simulink model "InvPendIdentPiMod2"  (R2025b)
settings: Solver=ode1  StartTime=0.0  StopTime=40  FixedStep=0.001  RelTol=1e-3
model workspace (MAT data in the model file):
  PID1D = 2
  PID1DD = 2
  PID1DI = 0.1
  PID1DP = 20
  PID1I = 0.1
  PID1P = 7
  PIDD = 2
  PIDDD = 2
  PIDDI = 0.1
  PIDDP = 7
  PIDI = 0.1
  PIDP = 20
undefined symbols (not defined in the file): magnitude, MQTTsample
libraries: simulink x6, slpidlib x4, raspberrypiCommlib x2, raspberrypiBasiclib x1, raspberrypiIOTlib x1
settings Model: SimulationMode=external  ExtModeTrigMode=oneshot  ExtModeTrigDuration=100000  Creator=Administrator  LastModifiedBy=brfon_9d4n8nc
settings SolverCC: AlgebraicLoopSolver=TrustRegion  PositivePriorityOrder=on  AutoInsertRateTranBlk=on
settings DataIOCC: SaveFormat=Array  SignalLoggingSaveFormat=ModelDataLogs  ReturnWorkspaceOutputs=off  SignalLoggingName=sigsOut
settings OptimizationCC: BlockReduction=off  BooleanDataType=off  EnhancedBackFolding=on  PassReuseOutputArgsAs=Individual arguments  ExpressionDepthLimit=2147483647.0  ZeroExternalMemoryAtStartup=off  ZeroInternalMemoryAtStartup=off  InitFltsAndDblsToZero=on  MaxStackSize=200000  OptimizeBlockOrder=speed  DifferentSizesBufferReuse=on  OptimizationCustomize=off  EfficientTunableParamExpr=on
settings DebuggingCC: SaveWithParameterizedLinksMsg=none  UnderspecifiedInitializationDetection=Classic  MergeDetectMultiDrivingBlocksExec=none  SignalResolutionControl=TryResolveAllWithWarning  MultiTaskDSMMsg=warning  ParameterTunabilityLossMsg=error  FcnCallInpInsideContextMsg=warning  UnconnectedInputMsg=warning  UnconnectedOutputMsg=warning  UnconnectedLineMsg=warning  AllowSymbolicDim=off  StateNameClashWarn=warning  SFUnexpectedBacktrackingDiag=warning  SFNoUnconditionalDefaultTransitionDiag=warning  SFExecutionAtInitializationDiag=none  ArithmeticOperatorsInVariantConditions=warning
settings HardwareCC: ProdBitPerLong=64.0  ProdLargestAtomicInteger=LongLong  ProdLargestAtomicFloat=Double  ProdLongLongMode=on  ProdHWDeviceType=ARM Compatible->ARM Cortex-A (64-bit)  TargetBitPerLong=64.0  TargetBitPerPointer=64.0  TargetIntDivRoundTo=Zero  TargetEndianess=LittleEndian  TargetWordSize=64.0  TargetHWDeviceType=Intel->x86-64
settings ModelReferenceCC: EnableRefExpFcnMdlSchedulingChecks=on  PropagateSignalLabelsOutOfModel=off
settings SFSimCC: SimUseLocalCustomCode=off  CustomCodeUndefinedFunction=UseInterfaceOnly
settings RTWCC: SystemTargetFile=ert.tlc  HardwareBoard=Raspberry Pi (64bit)  TLCOptions="-aInlineSetEventsForThisBaseRateFcn=TLC_FALSE -aSuppressMultiTaskScheduler=TLC_FALSE  -aRateBasedStepFcn=0"  TemplateMakefile=ert_default_tmf  RTWUseLocalCustomCode=off  Toolchain=GNU GCC Embedded Linux  BuildConfiguration=Faster Runs  GPUComputeCapability=3.5  Description=Embedded Coder
settings CodeAppCC: ForceParamTrailComments=on  IgnoreCustomStorageClasses=off  MaxIdLength=95.0  OperatorAnnotations=on  SimulinkDataObjDesc=on  SFDataObjDesc=on  InsertBlockDesc=on
settings ERTTargetCC: ExtModeTransport=2.0  ExtModeStaticAlloc=on  ExtModeMexFile=ext_xcp  ExtModeIntrfLevel=Level2 - Open  InlinedParameterPlacement=Hierarchical  CodeReplacementLibrary=ARM Cortex-A CMSIS  SupportContinuousTime=on  SupportVariableSizeSignals=on
settings ConfigComp: CovMetricSettings=dw  CovSaveCumulativeToWorkspaceVar=on  CovSaveSingleToWorkspaceVar=on  CovExternalEMLEnable=off

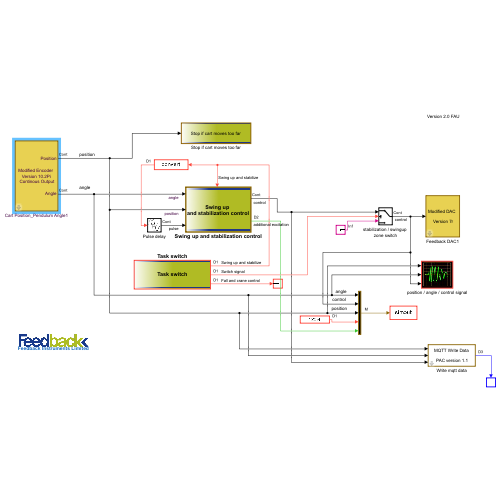
[thumbnail: Simulink's stored preview of the top-level diagram]
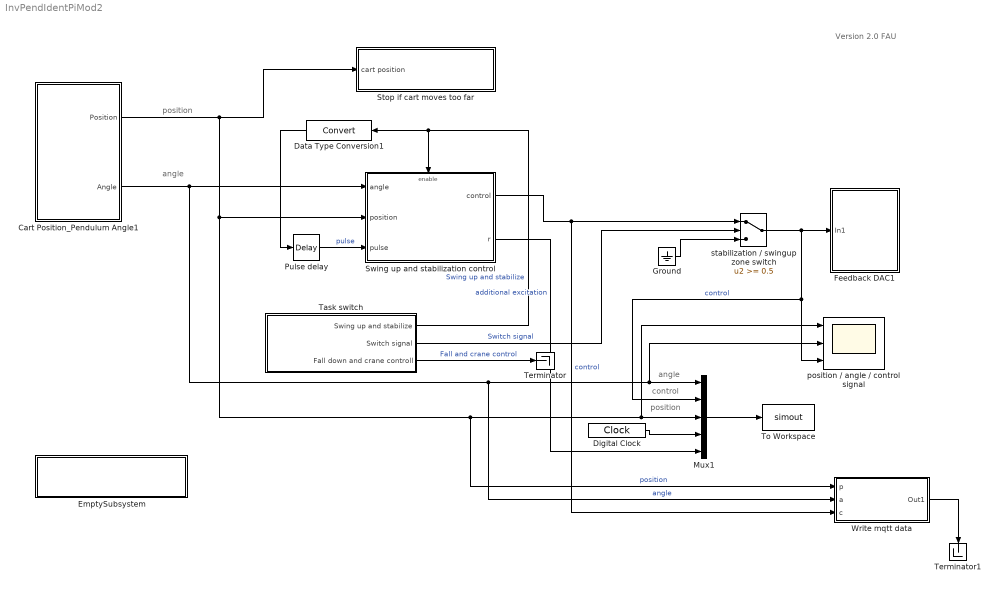
== system InvPendIdentPiMod2 ==
  note: position
  note: angle
  note: Version 2.0 FAU
  note: angle
  note: position
  note: control
  Cart Position_Pendulum Angle1 : Subsystem  mask(Feedback Encoder Block){st=0.001, of1=0, of2=-1024}
      mask prompts: st "Sample Time"; of1 "Channel 1 Offset"; of2 "Channel 2 Offset"
      mask help: Special block to use with the Feedback experiments to read encoder channels using the digital I/O lines
      mask Display:
      | %image(imread('bckg.bmp'))
      | disp('Modified Encoder \nVersion 10.2Pi\n Continous Output')
      | port_label('output', 1, 'Position')
      | port_label('output', 2, 'Angle')
  Data Type Conversion1 : DataTypeConversion  SaturateOnIntegerOverflow=off  RndMeth=Floor
  Digital Clock : DigitalClock  SampleTime=0.001
  EmptySubsystem : Subsystem
      mask Display:
      | image(imread('FB-inst-blue2.jpg'))
      | disp('\n\nFeedback Instruments Limited')
  Feedback DAC1 : Subsystem  mask(DAC Unit for Feedback Experiments){st=0.001, ch=1}
      mask prompts: st "Sample Time"; ch "Output Channel"
      mask help:
      | Digital to Analog Output  for Feedback Experiments
      | using Advantech PCI1711  I/O board
      mask Display:
      | %image(imread('bckg.bmp'))
      | disp('Modified DAC \n\n Version 7r')
  Ground : Ground
  Mux1 : Mux  Inputs=5
  Pulse delay : TransportDelay  DelayTime=0.3  FixedBuffer=on
  Stop if cart moves too far : Subsystem
      mask Display:
      | image(imread('bckg.bmp'))
      | disp('Stop if cart moves too far')
  Swing up and stabilization control : Subsystem  TreatAsAtomicUnit=on
      mask Display:
      | image(imread('bckg.bmp'))
      | disp('Swing up \nand stabilization control')
  Task switch : Subsystem
      mask Display:
      | image(imread('bckg.bmp'))
      | disp('Task switch')
  Terminator : Terminator
  Terminator1 : Terminator
  To Workspace : ToWorkspace  VariableName=simout  SampleTime=0.001
  Write mqtt data : Subsystem
      mask Display: disp('MQTT Write Data\n\n PAC version 1.1')
  position / angle / control signal : Scope  NumInputPorts=3
      settings: SampleTime=0.001  ActiveDisplayYMinimum=-0.55  ActiveDisplayYMaximum=0.35  DataLoggingMaxPoints=100000
      mask Display: image(imread('scope.jpg'))
  stabilization / swingup zone switch : Switch  Threshold=0.5  SaturateOnIntegerOverflow=off  InputSameDT=off
  wires:
  Cart Position_Pendulum Angle1/1(Position) -> Stop if cart moves too far/1(cart position), Write mqtt data/1(p), Mux1/3, position / angle / control signal/1, Swing up and stabilization control/2(position)  "position"
  Cart Position_Pendulum Angle1/2(Angle) -> Write mqtt data/2(a), Mux1/1, position / angle / control signal/2, Swing up and stabilization control/1(angle)  "angle"
  stabilization / swingup zone switch/1 -> Feedback DAC1/1(In1), Mux1/2, position / angle / control signal/3  "control"
  Swing up and stabilization control/1(control) -> Write mqtt data/3(c), stabilization / swingup zone switch/1  "control"
  Pulse delay/1 -> Swing up and stabilization control/3(pulse)  "pulse"
  Data Type Conversion1/1 -> Pulse delay/1
  Task switch/2(Switch signal) -> stabilization / swingup zone switch/2  "Switch signal"
  Mux1/1 -> To Workspace/1
  Task switch/3(Fall down and crane controll) -> Terminator/1  "Fall and crane control"
  Ground/1 -> stabilization / swingup zone switch/3
  Task switch/1(Swing up and stabilize) -> Data Type Conversion1/1, Swing up and stabilization control/Enable  "Swing up and stabilize"
  Digital Clock/1 -> Mux1/4
  Swing up and stabilization control/2(r) -> Mux1/5  "additional excitation"
  Write mqtt data/1(Out1) -> Terminator1/1

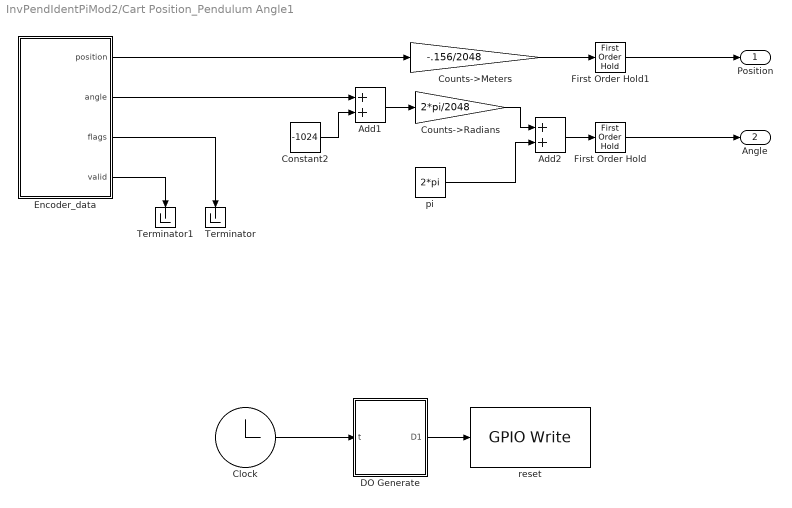
== system InvPendIdentPiMod2/Cart Position_Pendulum Angle1 ==
  Add1 : Sum
  Add2 : Sum
  Clock : Clock
  Constant2 : Constant  Value=-1024
  Counts->Meters : Gain  Gain=-.156/2048  SaturateOnIntegerOverflow=on  OutDataTypeStr=Inherit: Same as input  ParamDataTypeStr=Inherit: Same as input
  Counts->Radians : Gain  Gain=2*pi/2048  SaturateOnIntegerOverflow=on  OutDataTypeStr=Inherit: Same as input  ParamDataTypeStr=Inherit: Same as input
  DO Generate : MATLAB Function  TreatAsAtomicUnit=on
  Encoder_data : Subsystem
  First Order Hold : FirstOrderHold  OutputAlgorithm=Fast (Minimize Error)  ErrorTolerance=inf  AllowContinuousInput=on
  First Order Hold1 : FirstOrderHold  OutputAlgorithm=Fast (Minimize Error)  ErrorTolerance=inf  AllowContinuousInput=on
  Terminator : Terminator
  Terminator1 : Terminator
  pi : Constant  Value=2*pi
  reset : raspberrypiBasiclib/GPIO Write  BoardProperty=Pi 5 Model  gpio=6  blockPlatform=Raspberry Pi  PinNumber=17  board=[]  direction=[]
  Position : Outport
  Angle : Outport  Port=2
  wires:
  pi/1 -> Add2/2
  Counts->Radians/1 -> Add2/1
  Counts->Meters/1 -> First Order Hold1/1
  Clock/1 -> DO Generate/1(t)
  DO Generate/1(D1) -> reset/1
  Encoder_data/2(angle) -> Add1/1
  Encoder_data/1(position) -> Counts->Meters/1
  Add1/1 -> Counts->Radians/1
  Constant2/1 -> Add1/2
  Encoder_data/4(valid) -> Terminator1/1
  Encoder_data/3(flags) -> Terminator/1
  Add2/1 -> First Order Hold/1
  First Order Hold/1 -> Angle/1
  First Order Hold1/1 -> Position/1

== system InvPendIdentPiMod2/EmptySubsystem ==

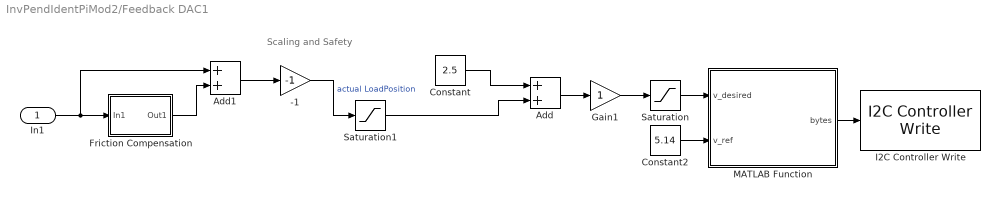
== system InvPendIdentPiMod2/Feedback DAC1 ==
  note: Scaling and Safety
  In1 : Inport
  -1 : Gain  Gain=-1  SaturateOnIntegerOverflow=on  OutDataTypeStr=Inherit: Same as input  ParamDataTypeStr=Inherit: Same as input
  Add : Sum  OutDataTypeStr=Inherit: Same as first input
  Add1 : Sum
  Constant : Constant  Value=2.5
  Constant2 : Constant  Value=5.14  SampleTime=-1
  Friction Compensation : Subsystem  mask(linear){frictionCompNeg=.1, frictionCompPos=.1}
      mask prompts: frictionCompNeg "Friction Compensation Magnitude in Negative Direction"; frictionCompPos "Friction Compensation Magnitude in Positive Direction"
      mask Display: plot(0,0,100,100,[40,30,20],[87,85,80],[46,54,54,46,46],[90,90,80,80,90],[46,45,45,46,54,55,55,54,46],[78,80,90,91,91,90,80,78,78],[51,51,49,49],[78,10,10,78],[90,80,70,60],[70,80,85,88],[20,10],[80,70],[20,20,15],[73,80,80],[85,80,80],[80,80,74])
  Gain1 : Gain
  I2C Controller Write : raspberrypiCommlib/I2C Controller Write  BoardProperty=Pi 5 Model  I2CModule=1  Mode=Master  SlaveAddress=0x60  SlaveByteOrder=BigEndian  Direction=Transmitter  RegisterAddressMode=off  RegisterAddress=0  SlaveDataType=uint8  DataLength=1  NoAck=off  RepeatedStart=off  OutputStatus=off
  MATLAB Function : MATLAB Function  TreatAsAtomicUnit=on
  Saturation : Saturate  UpperLimit=5.0  LowerLimit=0
  Saturation1 : Saturate  UpperLimit=2.5  LowerLimit=-2.5
  wires:
  Saturation1/1 -> Add/2
  Gain1/1 -> Saturation/1
  Add/1 -> Gain1/1
  Constant/1 -> Add/1
  Friction Compensation/1(Out1) -> Add1/2
  In1/1 -> Friction Compensation/1(In1), Add1/1
  -1/1 -> Saturation1/1  "actual LoadPosition"
  Add1/1 -> -1/1
  Constant2/1 -> MATLAB Function/2(v_ref)
  Saturation/1 -> MATLAB Function/1(v_desired)
  MATLAB Function/1(bytes) -> I2C Controller Write/1

== system InvPendIdentPiMod2/Stop if cart moves too far ==
  cart position : Inport
  Abs3 : Abs  SaturateOnIntegerOverflow=off
  Compare To Constant1 : simulink/Logic and Bit Operations/Compare To Constant  relop=>  const=0.4  OutDataTypeStr=boolean  ZeroCross=off
  Data Type Conversion1 : DataTypeConversion  SaturateOnIntegerOverflow=off  RndMeth=Floor
  Stop Simulation if cart moves to far : Stop
  wires:
  Abs3/1 -> Compare To Constant1/1
  Compare To Constant1/1 -> Data Type Conversion1/1
  Data Type Conversion1/1 -> Stop Simulation if cart moves to far/1
  cart position/1 -> Abs3/1

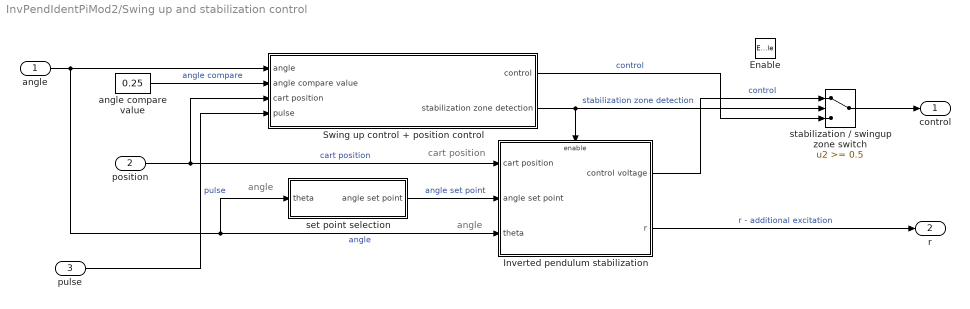
== system InvPendIdentPiMod2/Swing up and stabilization control ==
  note: angle
  note: cart position
  note: angle
  angle : Inport
  position : Inport  Port=2
  pulse : Inport  Port=3
  Enable : EnablePort
  Inverted pendulum stabilization : Subsystem  TreatAsAtomicUnit=on
      mask Display:
      | image(imread('bckg.bmp'))
      | disp('Inverted pendulum \nstabilization')
  Swing up control + position control : Subsystem
      mask Display:
      | image(imread('bckg.bmp'))
      | disp('Swing up control \nand position control')
  angle compare value : Constant  Value=0.25
  set point selection : Subsystem
      mask Display:
      | image(imread('bckg.bmp'))
      | disp('set point selection')
  stabilization / swingup zone switch : Switch  Threshold=0.5  SaturateOnIntegerOverflow=off  InputSameDT=off
  control : Outport
  r : Outport  Port=2
  wires:
  angle/1 -> Swing up control + position control/1(angle), set point selection/1(theta), Inverted pendulum stabilization/3(theta)  "angle"
  Swing up control + position control/1(control) -> stabilization / swingup zone switch/3  "control"
  Inverted pendulum stabilization/1(control voltage) -> stabilization / swingup zone switch/1  "control"
  set point selection/1(angle set point) -> Inverted pendulum stabilization/2(angle set point)  "angle set point"
  Swing up control + position control/2(stabilization zone detection) -> stabilization / swingup zone switch/2, Inverted pendulum stabilization/Enable  "stabilization zone detection"
  angle compare value/1 -> Swing up control + position control/2(angle compare value)  "angle compare"
  position/1 -> Inverted pendulum stabilization/1(cart position), Swing up control + position control/3(cart position)  "cart position"
  stabilization / swingup zone switch/1 -> control/1
  pulse/1 -> Swing up control + position control/4(pulse)  "pulse"
  Inverted pendulum stabilization/2(r) -> r/1  "r - additional excitation"

== system InvPendIdentPiMod2/Task switch ==
  Compare To Constant : simulink/Logic and Bit Operations/Compare To Constant  relop=<  const=0.5  OutDataTypeStr=boolean  ZeroCross=off
  Compare To Constant1 : simulink/Logic and Bit Operations/Compare To Constant  relop=>  const=0.5  OutDataTypeStr=boolean  ZeroCross=off
  Pulse Generator : DiscretePulseGenerator  PulseType=Time based  Period=60  PulseWidth=90
  Swing up and stabilize : Outport
  Switch signal : Outport  Port=2
  Fall down and crane controll : Outport  Port=3
  wires:
  Pulse Generator/1 -> Compare To Constant1/1, Switch signal/1, Compare To Constant/1
  Compare To Constant1/1 -> Swing up and stabilize/1
  Compare To Constant/1 -> Fall down and crane controll/1

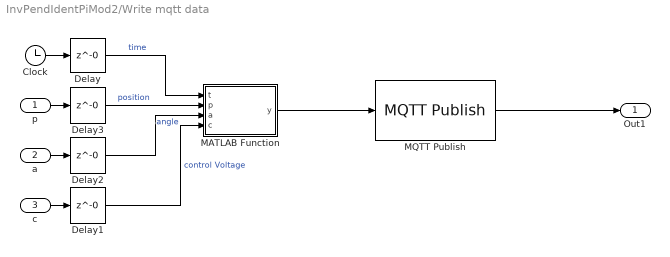
== system InvPendIdentPiMod2/Write mqtt data ==
  p : Inport
  a : Inport  Port=2
  c : Inport  Port=3
  Clock : Clock
  Delay{,1..3} (4 alike) : Delay  DelayLength=0  InitialCondition=0  SampleTime=MQTTsample
  MATLAB Function : MATLAB Function  TreatAsAtomicUnit=on
  MQTT Publish : raspberrypiIOTlib/MQTT Publish  Topic=raspi/to_django  QoS=0  RetainMsg=off  blockPlatform=RASPBERRYPI
  Out1 : Outport
  wires:
  MQTT Publish/1 -> Out1/1
  a/1 -> Delay2/1
  Clock/1 -> Delay/1
  Delay/1 -> MATLAB Function/1(t)  "time"
  p/1 -> Delay3/1
  Delay2/1 -> MATLAB Function/3(a)  "angle"
  c/1 -> Delay1/1
  Delay1/1 -> MATLAB Function/4(c)  "control Voltage"
  MATLAB Function/1(y) -> MQTT Publish/1
  Delay3/1 -> MATLAB Function/2(p)  "position"

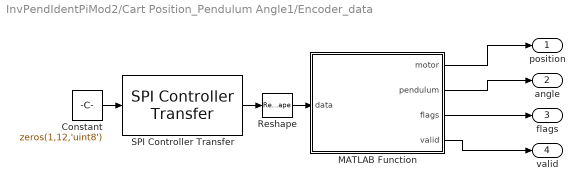
== system InvPendIdentPiMod2/Cart Position_Pendulum Angle1/Encoder_data ==
  Constant : Constant  Value=zeros(1,12,'uint8')
  MATLAB Function : MATLAB Function  TreatAsAtomicUnit=on
  Reshape : Reshape
  SPI Controller Transfer : raspberrypiCommlib/SPI Controller Transfer  BoardProperty=Pi 5 Model  SSPin=SPI0_CE0  SPIModule=uint32(0)  Mode=Master  BusSpeed=1000000  Pin=uint32(0)  FirstBitToTransfer=Most significant bit (MSB)  ClockMode=1  BlockFunction=Transfer  RegisterAddress=0  OutputDataType=int8  OutputDataLength=1
  position : Outport
  angle : Outport  Port=2
  flags : Outport  Port=3
  valid : Outport  Port=4
  wires:
  Constant/1 -> SPI Controller Transfer/1
  MATLAB Function/3(flags) -> flags/1
  SPI Controller Transfer/1 -> Reshape/1
  Reshape/1 -> MATLAB Function/1(data)
  MATLAB Function/2(pendulum) -> angle/1
  MATLAB Function/4(valid) -> valid/1
  MATLAB Function/1(motor) -> position/1

== system InvPendIdentPiMod2/Feedback DAC1/Friction Compensation ==
  In1 : Inport
  " " : Gain  Gain=frictionCompPos  SaturateOnIntegerOverflow=on  OutDataTypeStr=Inherit: Same as input  ParamDataTypeStr=Inherit: Same as input
  3 : Switch
  Gain3 : Gain  Gain=frictionCompNeg  SaturateOnIntegerOverflow=on  OutDataTypeStr=Inherit: Same as input  ParamDataTypeStr=Inherit: Same as input
  Sign2 : Signum  Tag=T
  Out1 : Outport  InitialOutput=0
  wires:
  In1/1 -> Sign2/1
  " "/1 -> 3/1
  Gain3/1 -> 3/3
  Sign2/1 -> Gain3/1, " "/1, 3/2
  3/1 -> Out1/1

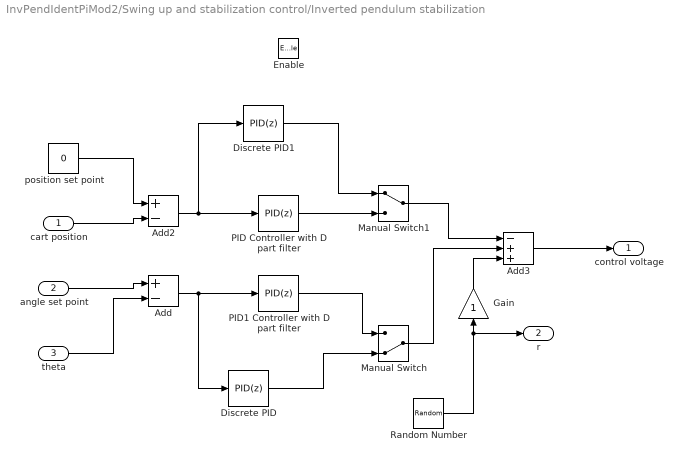
== system InvPendIdentPiMod2/Swing up and stabilization control/Inverted pendulum stabilization ==
  cart position : Inport
  angle set point : Inport  Port=2
  theta : Inport  Port=3
  Enable : EnablePort
  Add : Sum  Inputs=+-
  Add2 : Sum  Inputs=+-
  Add3 : Sum  Inputs=-++
  Discrete PID : slpidlib/PID Controller  Controller=PID  Form=Parallel  TimeDomain=Discrete-time  UseExternalTs=off  SampleTime=-1  IntegratorMethod=Forward Euler  FilterMethod=Forward Euler  ControllerParametersSource=internal  P=PIDP  I=PIDI  UseKiTs=off  D=PIDD  UseExternalDerivativeSource=off  N=100  UseFilter=on  TunerSelectOption=Transfer Function Based (PID Tuner App)  InitialConditionSource=internal  InitialConditionForIntegrator=0  InitialConditionForFilter=0  DifferentiatorICPrevScaledInput=0  ExternalReset=none  TrackingMode=off  Kt=1  LimitOutput=off  SatLimitsSource=internal  UpperSaturationLimit=inf  LowerSaturationLimit=-inf  LinearizeAsGain=on  AntiWindupMode=none  Kb=1  LimitIntegrator=off  UpperIntegratorSaturationLimit=inf  LowerIntegratorSaturationLimit=-inf  POutMin=[]  POutMax=[]  IOutMin=[]  IOutMax=[]  DOutMin=[]  DOutMax=[]  NOutMin=[]  NOutMax=[]  SumOutMin=[]  SumOutMax=[]  SaturationOutMin=[]  SaturationOutMax=[]  PParamMin=[]  PParamMax=[]  IParamMin=[]  IParamMax=[]  DParamMin=[]  DParamMax=[]  NParamMin=[]  NParamMax=[]  KbParamMin=[]  KbParamMax=[]  KtParamMin=[]  KtParamMax=[]  KbOutMin=[]  KbOutMax=[]  KtOutMin=[]  KtOutMax=[]  IntegratorOutMin=[]  IntegratorOutMax=[]  FilterOutMin=[]  FilterOutMax=[]  SumI1OutMin=[]  SumI1OutMax=[]  SumI2OutMin=[]  SumI2OutMax=[]  SumI3OutMin=[]  SumI3OutMax=[]  SumI4OutMin=[]  SumI4OutMax=[]  SumDOutMin=[]  SumDOutMax=[]  DifferentiatorOutMin=[]  DifferentiatorOutMax=[]  FilterDiffOutCoefMin=[]  FilterDiffOutCoefMax=[]  ReciprocalOutMin=[]  ReciprocalOutMax=[]  SumDenOutMin=[]  SumDenOutMax=[]  SumNumOutMin=[]  SumNumOutMax=[]  DivideOutMin=[]  DivideOutMax=[]  UdiffTsProdOutMin=[]  UdiffTsProdOutMax=[]  NTsProdOutMin=[]  NTsProdOutMax=[]  UintegralTsProdOutMin=[]  UintegralTsProdOutMax=[]  UngainTsProdOutMin=[]  UngainTsProdOutMax=[]  ClampingZeroOutDataTypeStr=Inherit: Inherit via back propagation  ClampingZeroOutMin=[]  ClampingZeroOutMax=[]  FilterDenConstantOutDataTypeStr=Inherit: Inherit via back propagation  FilterDenConstantOutMin=[]  FilterDenConstantOutMax=[]  PCopyOutDataTypeStr=Inherit: Inherit via back propagation  PCopyOutMin=[]  PCopyOutMax=[]  NCopyOutDataTypeStr=Inherit: Inherit via back propagation  NCopyOutMin=[]  NCopyOutMax=[]  IntegratorContinuousStateAttributes=''  IntegratorStateMustResolveToSignalObject=off  IntegratorRTWStateStorageClass=Auto  FilterContinuousStateAttributes=''  FilterStateMustResolveToSignalObject=off  FilterRTWStateStorageClass=Auto  ParallelPVariant=InternalParameters  IdealPVariant=Disabled  IVariant=InternalParameters  DVariant=InternalParameters  IntegratorVariant=Discrete  SatVariant=Disabled  AWVariant=Passthrough  PCopyVariant=Disabled  TRVariant=Disabled  FdbkBlocksVariant=Forward  IdealPFdbkVariant=Disabled  SatFdbkVariant=Disabled  DerivativeFilterVariant=ForwardEulerFilter  NVariant=InternalParameters  NCopyVariant=Disabled  FilterICVariant=InternalICsFilter  IntegratorICVariant=InternalICs  ExternalResetVariant=Disabled  TRSumVariant=Passthrough  SumFdbkVariant=Disabled  SumVariant=Sum_PID  TsampFilterVariant=InternalTs  TsampNgainVariant=Passthrough  TsampIntegralVariant=Disabled_SignalSpec  ExternalSaturationOutDataTypeStr=Inherit: Same as second input  DerivativeSourceVariant=ErrorSignal  PreIntVariant=InternalPreInt
  Discrete PID1 : slpidlib/PID Controller  Controller=PID  Form=Parallel  TimeDomain=Discrete-time  UseExternalTs=off  SampleTime=-1  IntegratorMethod=Forward Euler  FilterMethod=Forward Euler  ControllerParametersSource=internal  P=PID1P  I=PID1I  UseKiTs=off  D=PID1D  UseExternalDerivativeSource=off  N=100  UseFilter=on  TunerSelectOption=Transfer Function Based (PID Tuner App)  InitialConditionSource=internal  InitialConditionForIntegrator=0  InitialConditionForFilter=0  DifferentiatorICPrevScaledInput=0  ExternalReset=none  TrackingMode=off  Kt=1  LimitOutput=off  SatLimitsSource=internal  UpperSaturationLimit=inf  LowerSaturationLimit=-inf  LinearizeAsGain=on  AntiWindupMode=none  Kb=1  LimitIntegrator=off  UpperIntegratorSaturationLimit=inf  LowerIntegratorSaturationLimit=-inf  POutMin=[]  POutMax=[]  IOutMin=[]  IOutMax=[]  DOutMin=[]  DOutMax=[]  NOutMin=[]  NOutMax=[]  SumOutMin=[]  SumOutMax=[]  SaturationOutMin=[]  SaturationOutMax=[]  PParamMin=[]  PParamMax=[]  IParamMin=[]  IParamMax=[]  DParamMin=[]  DParamMax=[]  NParamMin=[]  NParamMax=[]  KbParamMin=[]  KbParamMax=[]  KtParamMin=[]  KtParamMax=[]  KbOutMin=[]  KbOutMax=[]  KtOutMin=[]  KtOutMax=[]  IntegratorOutMin=[]  IntegratorOutMax=[]  FilterOutMin=[]  FilterOutMax=[]  SumI1OutMin=[]  SumI1OutMax=[]  SumI2OutMin=[]  SumI2OutMax=[]  SumI3OutMin=[]  SumI3OutMax=[]  SumI4OutMin=[]  SumI4OutMax=[]  SumDOutMin=[]  SumDOutMax=[]  DifferentiatorOutMin=[]  DifferentiatorOutMax=[]  FilterDiffOutCoefMin=[]  FilterDiffOutCoefMax=[]  ReciprocalOutMin=[]  ReciprocalOutMax=[]  SumDenOutMin=[]  SumDenOutMax=[]  SumNumOutMin=[]  SumNumOutMax=[]  DivideOutMin=[]  DivideOutMax=[]  UdiffTsProdOutMin=[]  UdiffTsProdOutMax=[]  NTsProdOutMin=[]  NTsProdOutMax=[]  UintegralTsProdOutMin=[]  UintegralTsProdOutMax=[]  UngainTsProdOutMin=[]  UngainTsProdOutMax=[]  ClampingZeroOutDataTypeStr=Inherit: Inherit via back propagation  ClampingZeroOutMin=[]  ClampingZeroOutMax=[]  FilterDenConstantOutDataTypeStr=Inherit: Inherit via back propagation  FilterDenConstantOutMin=[]  FilterDenConstantOutMax=[]  PCopyOutDataTypeStr=Inherit: Inherit via back propagation  PCopyOutMin=[]  PCopyOutMax=[]  NCopyOutDataTypeStr=Inherit: Inherit via back propagation  NCopyOutMin=[]  NCopyOutMax=[]  IntegratorContinuousStateAttributes=''  IntegratorStateMustResolveToSignalObject=off  IntegratorRTWStateStorageClass=Auto  FilterContinuousStateAttributes=''  FilterStateMustResolveToSignalObject=off  FilterRTWStateStorageClass=Auto  ParallelPVariant=InternalParameters  IdealPVariant=Disabled  IVariant=InternalParameters  DVariant=InternalParameters  IntegratorVariant=Discrete  SatVariant=Disabled  AWVariant=Passthrough  PCopyVariant=Disabled  TRVariant=Disabled  FdbkBlocksVariant=Forward  IdealPFdbkVariant=Disabled  SatFdbkVariant=Disabled  DerivativeFilterVariant=ForwardEulerFilter  NVariant=InternalParameters  NCopyVariant=Disabled  FilterICVariant=InternalICsFilter  IntegratorICVariant=InternalICs  ExternalResetVariant=Disabled  TRSumVariant=Passthrough  SumFdbkVariant=Disabled  SumVariant=Sum_PID  TsampFilterVariant=InternalTs  TsampNgainVariant=Passthrough  TsampIntegralVariant=Disabled_SignalSpec  ExternalSaturationOutDataTypeStr=Inherit: Same as second input  DerivativeSourceVariant=ErrorSignal  PreIntVariant=InternalPreInt
  Gain : Gain
  Manual Switch : ManualSwitch  CurrentSetting=0
  Manual Switch1 : ManualSwitch
  PID Controller with D part filter : slpidlib/PID Controller  Controller=PID  Form=Parallel  TimeDomain=Discrete-time  UseExternalTs=off  SampleTime=-1  IntegratorMethod=Forward Euler  FilterMethod=Forward Euler  ControllerParametersSource=internal  P=PIDDP  I=PIDDI  UseKiTs=off  D=PIDDD  UseExternalDerivativeSource=off  N=100  UseFilter=on  TunerSelectOption=Transfer Function Based (PID Tuner App)  InitialConditionSource=internal  InitialConditionForIntegrator=0  InitialConditionForFilter=0  DifferentiatorICPrevScaledInput=0  ExternalReset=none  TrackingMode=off  Kt=1  LimitOutput=off  SatLimitsSource=internal  UpperSaturationLimit=inf  LowerSaturationLimit=-inf  LinearizeAsGain=on  AntiWindupMode=none  Kb=1  LimitIntegrator=off  UpperIntegratorSaturationLimit=inf  LowerIntegratorSaturationLimit=-inf  POutMin=[]  POutMax=[]  IOutMin=[]  IOutMax=[]  DOutMin=[]  DOutMax=[]  NOutMin=[]  NOutMax=[]  SumOutMin=[]  SumOutMax=[]  SaturationOutMin=[]  SaturationOutMax=[]  PParamMin=[]  PParamMax=[]  IParamMin=[]  IParamMax=[]  DParamMin=[]  DParamMax=[]  NParamMin=[]  NParamMax=[]  KbParamMin=[]  KbParamMax=[]  KtParamMin=[]  KtParamMax=[]  KbOutMin=[]  KbOutMax=[]  KtOutMin=[]  KtOutMax=[]  IntegratorOutMin=[]  IntegratorOutMax=[]  FilterOutMin=[]  FilterOutMax=[]  SumI1OutMin=[]  SumI1OutMax=[]  SumI2OutMin=[]  SumI2OutMax=[]  SumI3OutMin=[]  SumI3OutMax=[]  SumI4OutMin=[]  SumI4OutMax=[]  SumDOutMin=[]  SumDOutMax=[]  DifferentiatorOutMin=[]  DifferentiatorOutMax=[]  FilterDiffOutCoefMin=[]  FilterDiffOutCoefMax=[]  ReciprocalOutMin=[]  ReciprocalOutMax=[]  SumDenOutMin=[]  SumDenOutMax=[]  SumNumOutMin=[]  SumNumOutMax=[]  DivideOutMin=[]  DivideOutMax=[]  UdiffTsProdOutMin=[]  UdiffTsProdOutMax=[]  NTsProdOutMin=[]  NTsProdOutMax=[]  UintegralTsProdOutMin=[]  UintegralTsProdOutMax=[]  UngainTsProdOutMin=[]  UngainTsProdOutMax=[]  ClampingZeroOutDataTypeStr=Inherit: Inherit via back propagation  ClampingZeroOutMin=[]  ClampingZeroOutMax=[]  FilterDenConstantOutDataTypeStr=Inherit: Inherit via back propagation  FilterDenConstantOutMin=[]  FilterDenConstantOutMax=[]  PCopyOutDataTypeStr=Inherit: Inherit via back propagation  PCopyOutMin=[]  PCopyOutMax=[]  NCopyOutDataTypeStr=Inherit: Inherit via back propagation  NCopyOutMin=[]  NCopyOutMax=[]  IntegratorContinuousStateAttributes=''  IntegratorStateMustResolveToSignalObject=off  IntegratorRTWStateStorageClass=Auto  FilterContinuousStateAttributes=''  FilterStateMustResolveToSignalObject=off  FilterRTWStateStorageClass=Auto  ParallelPVariant=InternalParameters  IdealPVariant=Disabled  IVariant=InternalParameters  DVariant=InternalParameters  IntegratorVariant=Discrete  SatVariant=Disabled  AWVariant=Passthrough  PCopyVariant=Disabled  TRVariant=Disabled  FdbkBlocksVariant=Forward  IdealPFdbkVariant=Disabled  SatFdbkVariant=Disabled  DerivativeFilterVariant=ForwardEulerFilter  NVariant=InternalParameters  NCopyVariant=Disabled  FilterICVariant=InternalICsFilter  IntegratorICVariant=InternalICs  ExternalResetVariant=Disabled  TRSumVariant=Passthrough  SumFdbkVariant=Disabled  SumVariant=Sum_PID  TsampFilterVariant=InternalTs  TsampNgainVariant=Passthrough  TsampIntegralVariant=Disabled_SignalSpec  ExternalSaturationOutDataTypeStr=Inherit: Same as second input  DerivativeSourceVariant=ErrorSignal  PreIntVariant=InternalPreInt
  PID1 Controller with D part filter : slpidlib/PID Controller  Controller=PID  Form=Parallel  TimeDomain=Discrete-time  UseExternalTs=off  SampleTime=-1  IntegratorMethod=Forward Euler  FilterMethod=Forward Euler  ControllerParametersSource=internal  P=PID1DP  I=PID1DI  UseKiTs=off  D=PID1DD  UseExternalDerivativeSource=off  N=100  UseFilter=on  TunerSelectOption=Transfer Function Based (PID Tuner App)  InitialConditionSource=internal  InitialConditionForIntegrator=0  InitialConditionForFilter=0  DifferentiatorICPrevScaledInput=0  ExternalReset=none  TrackingMode=off  Kt=1  LimitOutput=off  SatLimitsSource=internal  UpperSaturationLimit=inf  LowerSaturationLimit=-inf  LinearizeAsGain=on  AntiWindupMode=none  Kb=1  LimitIntegrator=off  UpperIntegratorSaturationLimit=inf  LowerIntegratorSaturationLimit=-inf  POutMin=[]  POutMax=[]  IOutMin=[]  IOutMax=[]  DOutMin=[]  DOutMax=[]  NOutMin=[]  NOutMax=[]  SumOutMin=[]  SumOutMax=[]  SaturationOutMin=[]  SaturationOutMax=[]  PParamMin=[]  PParamMax=[]  IParamMin=[]  IParamMax=[]  DParamMin=[]  DParamMax=[]  NParamMin=[]  NParamMax=[]  KbParamMin=[]  KbParamMax=[]  KtParamMin=[]  KtParamMax=[]  KbOutMin=[]  KbOutMax=[]  KtOutMin=[]  KtOutMax=[]  IntegratorOutMin=[]  IntegratorOutMax=[]  FilterOutMin=[]  FilterOutMax=[]  SumI1OutMin=[]  SumI1OutMax=[]  SumI2OutMin=[]  SumI2OutMax=[]  SumI3OutMin=[]  SumI3OutMax=[]  SumI4OutMin=[]  SumI4OutMax=[]  SumDOutMin=[]  SumDOutMax=[]  DifferentiatorOutMin=[]  DifferentiatorOutMax=[]  FilterDiffOutCoefMin=[]  FilterDiffOutCoefMax=[]  ReciprocalOutMin=[]  ReciprocalOutMax=[]  SumDenOutMin=[]  SumDenOutMax=[]  SumNumOutMin=[]  SumNumOutMax=[]  DivideOutMin=[]  DivideOutMax=[]  UdiffTsProdOutMin=[]  UdiffTsProdOutMax=[]  NTsProdOutMin=[]  NTsProdOutMax=[]  UintegralTsProdOutMin=[]  UintegralTsProdOutMax=[]  UngainTsProdOutMin=[]  UngainTsProdOutMax=[]  ClampingZeroOutDataTypeStr=Inherit: Inherit via back propagation  ClampingZeroOutMin=[]  ClampingZeroOutMax=[]  FilterDenConstantOutDataTypeStr=Inherit: Inherit via back propagation  FilterDenConstantOutMin=[]  FilterDenConstantOutMax=[]  PCopyOutDataTypeStr=Inherit: Inherit via back propagation  PCopyOutMin=[]  PCopyOutMax=[]  NCopyOutDataTypeStr=Inherit: Inherit via back propagation  NCopyOutMin=[]  NCopyOutMax=[]  IntegratorContinuousStateAttributes=''  IntegratorStateMustResolveToSignalObject=off  IntegratorRTWStateStorageClass=Auto  FilterContinuousStateAttributes=''  FilterStateMustResolveToSignalObject=off  FilterRTWStateStorageClass=Auto  ParallelPVariant=InternalParameters  IdealPVariant=Disabled  IVariant=InternalParameters  DVariant=InternalParameters  IntegratorVariant=Discrete  SatVariant=Disabled  AWVariant=Passthrough  PCopyVariant=Disabled  TRVariant=Disabled  FdbkBlocksVariant=Forward  IdealPFdbkVariant=Disabled  SatFdbkVariant=Disabled  DerivativeFilterVariant=ForwardEulerFilter  NVariant=InternalParameters  NCopyVariant=Disabled  FilterICVariant=InternalICsFilter  IntegratorICVariant=InternalICs  ExternalResetVariant=Disabled  TRSumVariant=Passthrough  SumFdbkVariant=Disabled  SumVariant=Sum_PID  TsampFilterVariant=InternalTs  TsampNgainVariant=Passthrough  TsampIntegralVariant=Disabled_SignalSpec  ExternalSaturationOutDataTypeStr=Inherit: Same as second input  DerivativeSourceVariant=ErrorSignal  PreIntVariant=InternalPreInt
  Random Number : RandomNumber  Variance=0.3  Seed=425745685  SampleTime=0.05
  position set point : Constant  Value=0
  control voltage : Outport
  r : Outport  Port=2
  wires:
  Add/1 -> Discrete PID/1, PID1 Controller with D part filter/1
  position set point/1 -> Add2/1
  Add2/1 -> PID Controller with D part filter/1, Discrete PID1/1
  cart position/1 -> Add2/2
  theta/1 -> Add/2
  angle set point/1 -> Add/1
  Add3/1 -> control voltage/1
  Random Number/1 -> r/1, Gain/1
  Manual Switch/1 -> Add3/2
  PID1 Controller with D part filter/1 -> Manual Switch/1
  Discrete PID/1 -> Manual Switch/2
  Gain/1 -> Add3/3
  PID Controller with D part filter/1 -> Manual Switch1/2
  Manual Switch1/1 -> Add3/1
  Discrete PID1/1 -> Manual Switch1/1

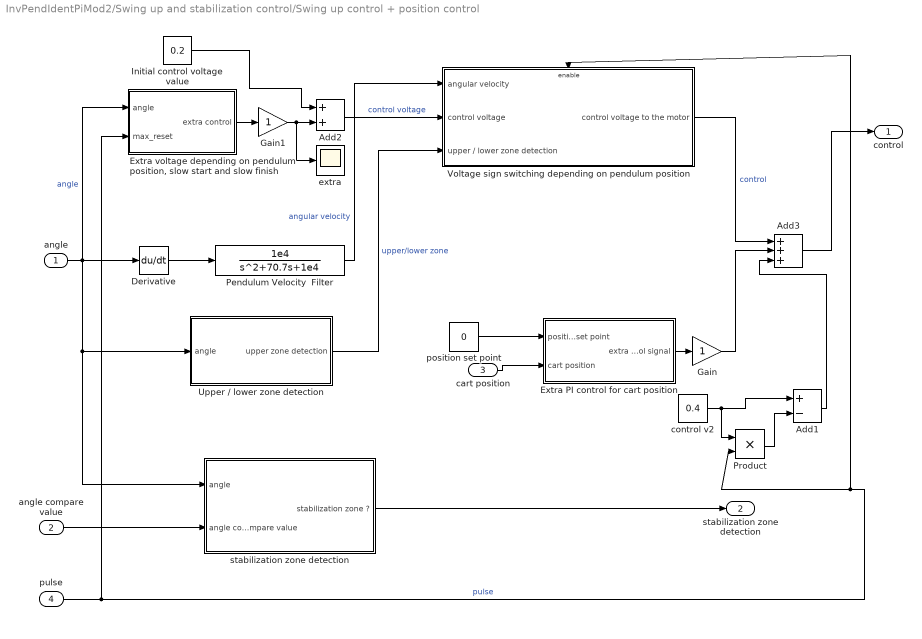
== system InvPendIdentPiMod2/Swing up and stabilization control/Swing up control + position control ==
  angle : Inport
  angle compare value : Inport  Port=2
  cart position : Inport  Port=3
  pulse : Inport  Port=4
  Add1 : Sum  Inputs=+-
  Add2 : Sum
  Add3 : Sum  Inputs=+++
  Derivative : Derivative
  Extra PI control for cart position : Subsystem
  "Extra voltage depending on pendulum position, slow start and slow finish" : Subsystem
      mask Display:
      | image(imread('bckg.bmp'))
      | disp('Extra voltage')
  Gain : Gain
  Gain1 : Gain
  Initial control voltage value : Constant  Value=0.2
  Pendulum Velocity  Filter : TransferFcn  Numerator=[1e4]  Denominator=[1 70.7 1e4]
  Product : Product  RndMeth=Zero
  Upper / lower zone detection : Subsystem
      mask Display:
      | image(imread('bckg.bmp'))
      | disp('Upper / lower zone \ndetection')
  Voltage sign switching depending on pendulum position : Subsystem
      mask Display:
      | image(imread('bckg.bmp'))
      | disp('Voltage sign switching depending on \npendulum position')
  control v2 : Constant  Value=0.4
  extra : Scope
      settings: SampleTime=0.05  TimeSpan=200  ActiveDisplayYMinimum=0  ActiveDisplayYMaximum=0.2  DataLoggingMaxPoints=50000  DataLoggingVariableName=ScopeData3
      mask Display: image(imread('scope.jpg'))
  position set point : Constant  Value=0
  "stabilization zone detection " : Subsystem
      mask Display:
      | image(imread('bckg.bmp'))
      | disp('stabilization zone detection')
  control : Outport
  stabilization zone detection : Outport  Port=2
  wires:
  Upper / lower zone detection/1(upper zone detection) -> Voltage sign switching depending on pendulum position/3(upper / lower zone detection)  "upper/lower zone"
  Initial control voltage value/1 -> Add2/1
  Add2/1 -> Voltage sign switching depending on pendulum position/2(control voltage)  "control voltage"
  angle/1 -> "Extra voltage depending on pendulum position, slow start and slow finish"/1(angle), Derivative/1, Upper / lower zone detection/1(angle), "stabilization zone detection "/1(angle)  "angle"
  Derivative/1 -> Pendulum Velocity  Filter/1
  Pendulum Velocity  Filter/1 -> Voltage sign switching depending on pendulum position/1(angular velocity)  "angular velocity"
  "stabilization zone detection "/1(stabilization zone ?) -> stabilization zone detection/1
  angle compare value/1 -> "stabilization zone detection "/2(angle compare value)
  position set point/1 -> Extra PI control for cart position/1(position set point)
  cart position/1 -> Extra PI control for cart position/2(cart position)
  Extra PI control for cart position/1(extra control signal) -> Gain/1
  Voltage sign switching depending on pendulum position/1(control voltage to the motor) -> Add3/1  "control"
  Add3/1 -> control/1
  Gain/1 -> Add3/2
  "Extra voltage depending on pendulum position, slow start and slow finish"/1(extra control) -> Gain1/1
  Gain1/1 -> Add2/2, extra/1
  pulse/1 -> Product/2, Voltage sign switching depending on pendulum position/Enable, "Extra voltage depending on pendulum position, slow start and slow finish"/2(max_reset)  "pulse"
  Add1/1 -> Add3/3
  control v2/1 -> Add1/1, Product/1
  Product/1 -> Add1/2

== system InvPendIdentPiMod2/Swing up and stabilization control/set point selection ==
  theta : Inport
  0 : Constant  Value=0
  2*pi : Constant  Value=2*pi
  Abs : Abs  SaturateOnIntegerOverflow=off
  zero velocity : Switch  Threshold=pi  SaturateOnIntegerOverflow=off  InputSameDT=off
  angle set point : Outport
  wires:
  zero velocity/1 -> angle set point/1
  theta/1 -> Abs/1
  Abs/1 -> zero velocity/2
  2*pi/1 -> zero velocity/1
  0/1 -> zero velocity/3

== system InvPendIdentPiMod2/Swing up and stabilization control/Swing up control + position control/Extra PI control for cart position ==
  position set point : Inport
  cart position : Inport  Port=2
  Add1 : Sum  Inputs=+-
  PID Controller with D part filter : Subsystem  AncestorBlock=simulink_extras/Additional Linear/PID Controller  mask(PID Controller){P=0.5, I=0.2, D=0}
      mask prompts: P "Proportional:"; I "Integral:"; D "Derivative:"
      mask help:
      | Enter expressions for proportional, integral, and derivative terms.
      | P+I/s+Ds
      mask Help: This block implements a PID controller where parameters are entered for the Proportional, Integral and Derivative terms. Unmask this block to see how it works. The derivative term is implemented using a true derivative block.
      mask Display:
      | image(imread('bckg.bmp'))
      | disp('PID')
  extra control signal : Outport
  wires:
  Add1/1 -> PID Controller with D part filter/1(In_1)
  position set point/1 -> Add1/1
  PID Controller with D part filter/1(Out_1) -> extra control signal/1
  cart position/1 -> Add1/2

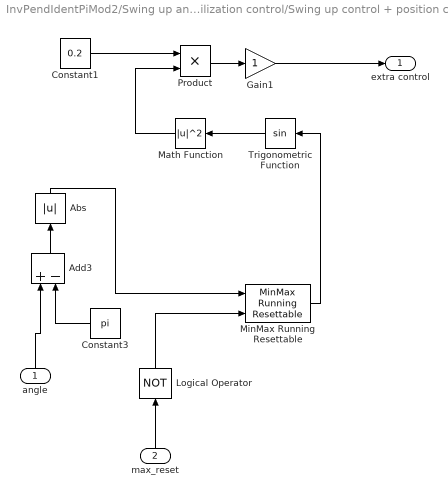
== system InvPendIdentPiMod2/Swing up and stabilization control/Swing up control + position control/Extra voltage depending on pendulum position, slow start and slow finish ==
  angle : Inport
  max_reset : Inport  Port=2
  Abs : Abs  SaturateOnIntegerOverflow=off
  Add3 : Sum  Inputs=+-
  Constant1 : Constant  Value=0.2
  Constant3 : Constant  Value=pi
  Gain1 : Gain
  Logical Operator : Logic  Operator=NOT  AllPortsSameDT=off  OutDataTypeStr=boolean
  Math Function : Math  Operator=magnitude^2  SignedPower=on
  MinMax Running Resettable : simulink/Math Operations/MinMax Running Resettable  Function=max  vinit=0.0
  Product : Product  RndMeth=Zero
  Trigonometric Function : Trigonometry
  extra control : Outport
  wires:
  Product/1 -> Gain1/1
  Constant1/1 -> Product/1
  Constant3/1 -> Add3/2
  Add3/1 -> Abs/1
  Abs/1 -> MinMax Running Resettable/1
  Trigonometric Function/1 -> Math Function/1
  Gain1/1 -> extra control/1
  Math Function/1 -> Product/2
  angle/1 -> Add3/1
  max_reset/1 -> Logical Operator/1
  MinMax Running Resettable/1 -> Trigonometric Function/1
  Logical Operator/1 -> MinMax Running Resettable/2

== system InvPendIdentPiMod2/Swing up and stabilization control/Swing up control + position control/Upper // lower zone detection ==
  angle : Inport
  Compare To Constant : simulink/Logic and Bit Operations/Compare To Constant  relop=<=  const=pi/2  OutDataTypeStr=uint8  ZeroCross=off
  Compare To Constant1 : simulink/Logic and Bit Operations/Compare To Constant  relop=>=  const=pi/2+pi  OutDataTypeStr=uint8  ZeroCross=off
  Logical Operator : Logic  Operator=OR  AllPortsSameDT=off  OutDataTypeStr=boolean
  upper zone detection : Outport
  wires:
  Compare To Constant/1 -> Logical Operator/1
  Compare To Constant1/1 -> Logical Operator/2
  angle/1 -> Compare To Constant/1, Compare To Constant1/1
  Logical Operator/1 -> upper zone detection/1

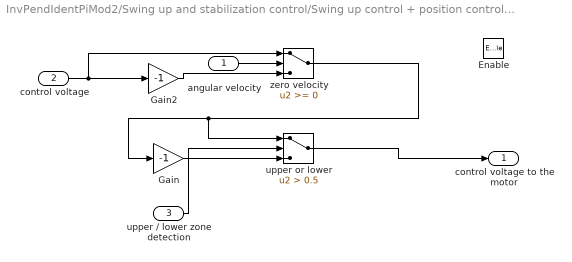
== system InvPendIdentPiMod2/Swing up and stabilization control/Swing up control + position control/Voltage sign switching depending on pendulum position ==
  angular velocity : Inport
  control voltage : Inport  Port=2
  upper / lower zone detection : Inport  Port=3
  Enable : EnablePort
  Gain : Gain  Gain=-1
  Gain2 : Gain  Gain=-1
  upper or lower : Switch  Criteria=u2 > Threshold  Threshold=0.5  SaturateOnIntegerOverflow=off  InputSameDT=off
  zero velocity : Switch  SaturateOnIntegerOverflow=off  InputSameDT=off
  control voltage to the motor : Outport
  wires:
  Gain/1 -> upper or lower/3
  zero velocity/1 -> upper or lower/1, Gain/1
  control voltage/1 -> zero velocity/1, Gain2/1
  Gain2/1 -> zero velocity/3
  angular velocity/1 -> zero velocity/2
  upper or lower/1 -> control voltage to the motor/1
  upper / lower zone detection/1 -> upper or lower/2

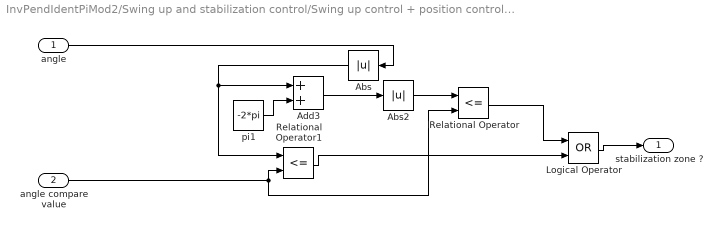
== system InvPendIdentPiMod2/Swing up and stabilization control/Swing up control + position control/stabilization zone detection  ==
  angle : Inport
  angle compare value : Inport  Port=2
  Abs : Abs  SaturateOnIntegerOverflow=off
  Abs2 : Abs  SaturateOnIntegerOverflow=off
  Add3 : Sum
  Logical Operator : Logic  Operator=OR  AllPortsSameDT=off  OutDataTypeStr=boolean
  Relational Operator : RelationalOperator  Operator=<=  OutDataTypeStr=boolean  InputSameDT=off
  Relational Operator1 : RelationalOperator  Operator=<=  OutDataTypeStr=boolean  InputSameDT=off
  pi1 : Constant  Value=-2*pi
  stabilization zone ? : Outport
  wires:
  Abs/1 -> Add3/1, Relational Operator1/1
  Relational Operator1/1 -> Logical Operator/2
  pi1/1 -> Add3/2
  Add3/1 -> Abs2/1
  Relational Operator/1 -> Logical Operator/1
  Abs2/1 -> Relational Operator/1
  angle/1 -> Abs/1
  Logical Operator/1 -> stabilization zone ?/1
  angle compare value/1 -> Relational Operator1/2, Relational Operator/2

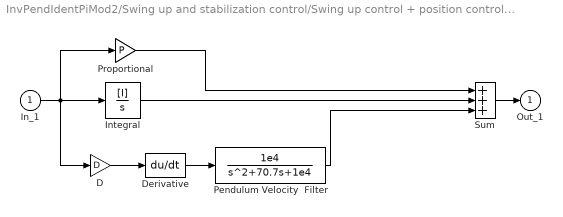
== system InvPendIdentPiMod2/Swing up and stabilization control/Swing up control + position control/Extra PI control for cart position/PID Controller with D part filter ==
  In_1 : Inport
  D : Gain  Gain=D  SaturateOnIntegerOverflow=on  OutDataTypeStr=Inherit: Same as input  ParamDataTypeStr=Inherit: Same as input
  Derivative : Derivative
  Integral : TransferFcn  Numerator=[I]  Denominator=[1 0]
  Pendulum Velocity  Filter : TransferFcn  Numerator=[1e4]  Denominator=[1 70.7 1e4]
  Proportional : Gain  Gain=P  SaturateOnIntegerOverflow=on  OutDataTypeStr=Inherit: Same as input  ParamDataTypeStr=Inherit: Same as input
  Sum : Sum  Inputs=+++  InputSameDT=on  SaturateOnIntegerOverflow=on  OutDataTypeStr=Inherit: Same as first input
  Out_1 : Outport  InitialOutput=0
  wires:
  Proportional/1 -> Sum/1
  Integral/1 -> Sum/2
  Derivative/1 -> Pendulum Velocity  Filter/1
  In_1/1 -> Integral/1, Proportional/1, D/1
  Sum/1 -> Out_1/1
  D/1 -> Derivative/1
  Pendulum Velocity  Filter/1 -> Sum/3

== matlab function InvPendIdentPiMod2/Feedback DAC1/MATLAB Function ==
  data: v_desired input; bytes output; v_ref input
function bytes = voltToMCP4725(v_desired, v_ref)
    % v_desired: desired output voltage (0 to v_ref)
    % v_ref: DAC supply voltage (5.0)
    dacVal = uint16(round((v_desired / v_ref) * 4095));
    dacVal = min(dacVal, uint16(4095));
    b0 = uint8(64);                        % 0x40 command byte
    b1 = uint8(bitshift(dacVal, -4));      % upper 8 bits
    b2 = uint8(bitshift(bitand(dacVal, uint16(15)), 4)); % lower 4 bits
    bytes = [b0; b1; b2];
end

== matlab function InvPendIdentPiMod2/Cart Position_Pendulum Angle1/DO Generate ==
  data: D1 output; t input
%%pendulum 10
function D1  = generate_DO(t)
    if t <= 0.002
        D1 = 1;  % RESET on first sample
    else
        D1 = 0;
    end
end



%%pendulum 5
% function [D1, D2] = generate_DO(counter, t)
%     if t <= 0.002
%         D1 = 1;  % RESET on first sample
%         % D2 = 0;
%     else
%         D1 = 0;
%     %     D2 = 0;
%         % if mod(counter, 4) < 2
%         %     D1 = 0;
%         %     D2 = 0;
%         % else
%         %     D1 = 1;
%         %     D2 = 0;
%         % end
%     end
% end


%%pendulum 4
% function DO = generate_DO(counter)
%     switch counter
%         case 0
%             DO = 4;  % Reset/idle
%         case 1
%             DO = 1;  % Set DO=1 (ESP32 prepares high byte)
%         case 2
%             DO = 4;  % Keep DO=1 (Simulink reads high byte)        
%         case 3
%             DO = 4;  % Keep DO=1 (Simulink reads high byte)        
%         case 4
%             DO = 2;  % Keep DO=1 (Simulink reads high byte)        
% %         case 3
% %             DO = 1;  % Keep DO=1 (Simulink reads high byte)
% %         case 3
% %             DO = 2; %seperations
% %         case 5
% %             DO = 4; %seperations
% %         case 4
% %             DO = 2;  % Set DO=2 (ESP32 prepares low byte)
% %         case 7
% %             DO = 2;  % Keep DO=2 (Simulink reads low byte)
% %         case 8
% %             DO = 2;  % Keep DO=2 (Simulink reads low byte)
% %         case 9
% %             DO = 4;  % Unlatch
%         otherwise
%             DO = 4;
%     end
% end
% 
% function DO = generate_DO(counter)
%     % Just toggle between 0 and 1
%     if counter == 0
%         DO = 1;  % Motor state
%     else
%         DO = 0;  % Pendulum state
%     end
% end

== matlab function InvPendIdentPiMod2/Write mqtt data/MATLAB Function ==
  data: t input; p input; y output; a input; c input
function y = fmtstr(t,p,a,c)

y = "{time: "+string(t)+", position: "+string(p)+", angle: "+string(a)+", control: "+string(c)+"}";

== matlab function InvPendIdentPiMod2/Cart Position_Pendulum Angle1/Encoder_data/MATLAB Function ==
  data: data input uint8 size=[1 12]; motor output; pendulum output; flags output; valid output
function [motor, pendulum, flags, valid] = unpack_spi(data)

% Checksum
chk = uint8(0);
for i = 1:9
    chk = bitxor(chk, data(i));
end
valid = logical(chk == data(10));

% Motor — bytes 1-4 little-endian
motor_int = int32(data(1)) + ...
        bitshift(int32(data(2)), 8) + ...
        bitshift(int32(data(3)), 16) + ...
        bitshift(int32(data(4)), 24);

% Pendulum — bytes 5-8 little-endian
pend_int = int32(data(5)) + ...
           bitshift(int32(data(6)), 8) + ...
           bitshift(int32(data(7)), 16) + ...
           bitshift(int32(data(8)), 24);

% Flags
flags = uint8(data(9));

% Output as single (32-bit float) for use in control blocks
motor    = double(motor_int);
pendulum = single(pend_int);

end
